simulink model "atlas_wheel_speed_loop"  (R2025a)
settings: Solver=ode23t  StartTime=0.0  StopTime=2  MaxStep=1e-3  RelTol=1e-3
model workspace (MAT data in the model file):
  Ass = [-4000  -3  0; 32088.2852292  -0.713073005093  0; 0  0.00666666666667  0]
  Bss = [666.666666667  0; 0  -67911.7147708; 0  0]
  Css = [0  0.00666666666667  0; 0  0  1]
  Dss = [0  0; 0  0]
  Ki = 15.9929267511
  Kp = 0.475908649842
  T_ramp = 0.0453859092535
  Ts = 0.01
  Vb = 7.4
  q_ang = 0.000872664625997
  w_ref = 6.15384615385
libraries: slpidlib x1, simulink x1
settings Model: Creator=mdsazzadhossain  LastModifiedBy=mdsazzadhossain

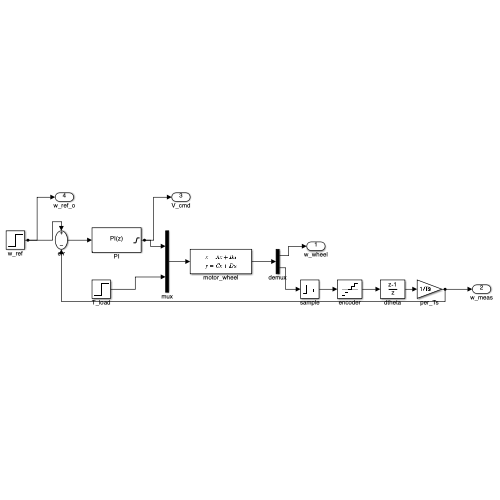
[thumbnail: Simulink's stored preview of the top-level diagram]
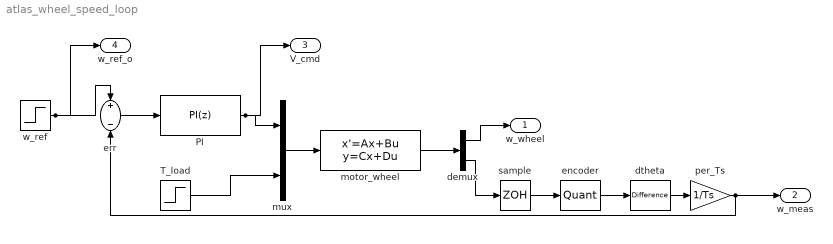
== system atlas_wheel_speed_loop ==
  PI : slpidlib/PID Controller  Controller=PI  Form=Parallel  TimeDomain=Discrete-time  UseExternalTs=off  SampleTime=Ts  IntegratorMethod=Forward Euler  FilterMethod=Forward Euler  ControllerParametersSource=internal  P=Kp  I=Ki  UseKiTs=off  D=0  UseExternalDerivativeSource=off  N=100  UseFilter=on  TunerSelectOption=Transfer Function Based (PID Tuner App)  InitialConditionSource=internal  InitialConditionForIntegrator=0  InitialConditionForFilter=0  DifferentiatorICPrevScaledInput=0  ExternalReset=none  TrackingMode=off  Kt=1  LimitOutput=on  SatLimitsSource=internal  UpperSaturationLimit=Vb  LowerSaturationLimit=-Vb  LinearizeAsGain=off  AntiWindupMode=clamping  Kb=1  LimitIntegrator=off  UpperIntegratorSaturationLimit=inf  LowerIntegratorSaturationLimit=-inf  POutMin=[]  POutMax=[]  IOutMin=[]  IOutMax=[]  DOutMin=[]  DOutMax=[]  NOutMin=[]  NOutMax=[]  SumOutMin=[]  SumOutMax=[]  SaturationOutMin=[]  SaturationOutMax=[]  PParamMin=[]  PParamMax=[]  IParamMin=[]  IParamMax=[]  DParamMin=[]  DParamMax=[]  NParamMin=[]  NParamMax=[]  KbParamMin=[]  KbParamMax=[]  KtParamMin=[]  KtParamMax=[]  KbOutMin=[]  KbOutMax=[]  KtOutMin=[]  KtOutMax=[]  IntegratorOutMin=[]  IntegratorOutMax=[]  FilterOutMin=[]  FilterOutMax=[]  SumI1OutMin=[]  SumI1OutMax=[]  SumI2OutMin=[]  SumI2OutMax=[]  SumI3OutMin=[]  SumI3OutMax=[]  SumI4OutMin=[]  SumI4OutMax=[]  SumDOutMin=[]  SumDOutMax=[]  DifferentiatorOutMin=[]  DifferentiatorOutMax=[]  FilterDiffOutCoefMin=[]  FilterDiffOutCoefMax=[]  ReciprocalOutMin=[]  ReciprocalOutMax=[]  SumDenOutMin=[]  SumDenOutMax=[]  SumNumOutMin=[]  SumNumOutMax=[]  DivideOutMin=[]  DivideOutMax=[]  UdiffTsProdOutMin=[]  UdiffTsProdOutMax=[]  NTsProdOutMin=[]  NTsProdOutMax=[]  UintegralTsProdOutMin=[]  UintegralTsProdOutMax=[]  UngainTsProdOutMin=[]  UngainTsProdOutMax=[]  ClampingZeroOutDataTypeStr=Inherit: Inherit via back propagation  ClampingZeroOutMin=[]  ClampingZeroOutMax=[]  FilterDenConstantOutDataTypeStr=Inherit: Inherit via back propagation  FilterDenConstantOutMin=[]  FilterDenConstantOutMax=[]  PCopyOutDataTypeStr=Inherit: Inherit via back propagation  PCopyOutMin=[]  PCopyOutMax=[]  NCopyOutDataTypeStr=Inherit: Inherit via back propagation  NCopyOutMin=[]  NCopyOutMax=[]  IntegratorContinuousStateAttributes=''  IntegratorStateMustResolveToSignalObject=off  IntegratorRTWStateStorageClass=Auto  FilterContinuousStateAttributes=''  FilterStateMustResolveToSignalObject=off  FilterRTWStateStorageClass=Auto  ParallelPVariant=InternalParameters  IdealPVariant=Disabled  IVariant=InternalParameters  DVariant=Disabled  IntegratorVariant=Discrete  SatVariant=Enabled  AWVariant=DiscClampingParallel  PCopyVariant=Disabled  TRVariant=Disabled  FdbkBlocksVariant=Forward  IdealPFdbkVariant=Disabled  SatFdbkVariant=Disabled  DerivativeFilterVariant=Disabled  NVariant=Disabled  NCopyVariant=Disabled_SignalSpec  FilterICVariant=Disabled  IntegratorICVariant=InternalICs  ExternalResetVariant=Disabled  TRSumVariant=Passthrough  SumFdbkVariant=Disabled  SumVariant=Sum_PI  TsampFilterVariant=InternalTs  TsampNgainVariant=Passthrough  TsampIntegralVariant=Disabled_SignalSpec  ExternalSaturationOutDataTypeStr=Inherit: Same as second input  DerivativeSourceVariant=Disabled  PreIntVariant=InternalPreInt
      settings: LibrarySourceBlock=simulink/Discrete/Discrete PID Controller
  T_load : Step  Time=1.0  After=T_ramp  SampleTime=0
  demux : Demux  Outputs=2
  dtheta : simulink/Discrete/Difference  ICPrevInput=0.0  OutMin=[]  OutMax=[]  OutDataType=fixdt(1, 16)  OutScaling=2^-10  DoSatur=off
  encoder : Quantizer  QuantizationInterval=q_ang
  err : Sum  Inputs=+-
  motor_wheel : StateSpace  A=Ass  B=Bss  C=Css  D=Dss  InitialCondition=0
  mux : Mux  Inputs=2
  per_Ts : Gain  Gain=1/Ts
  sample : ZeroOrderHold  SampleTime=Ts
  w_ref : Step  Time=0.1  After=w_ref  SampleTime=Ts
  w_wheel : Outport
  w_meas : Outport  Port=2
  V_cmd : Outport  Port=3
  w_ref_o : Outport  Port=4
  wires:
  w_ref/1 -> err/1, w_ref_o/1
  err/1 -> PI/1
  PI/1 -> mux/1, V_cmd/1
  T_load/1 -> mux/2
  mux/1 -> motor_wheel/1
  motor_wheel/1 -> demux/1
  demux/1 -> w_wheel/1
  demux/2 -> sample/1
  sample/1 -> encoder/1
  encoder/1 -> dtheta/1
  dtheta/1 -> per_Ts/1
  per_Ts/1 -> w_meas/1, err/2
